simulink model "can2_comp_cmd_unpack"  (R2026b)
settings: Solver=VariableStepAuto
undefined symbols (not defined in the file or in its folder): P
libraries: simulink x1, svdutilitieslib x1
settings Model: Creator=aomar  LastModifiedBy=aomar

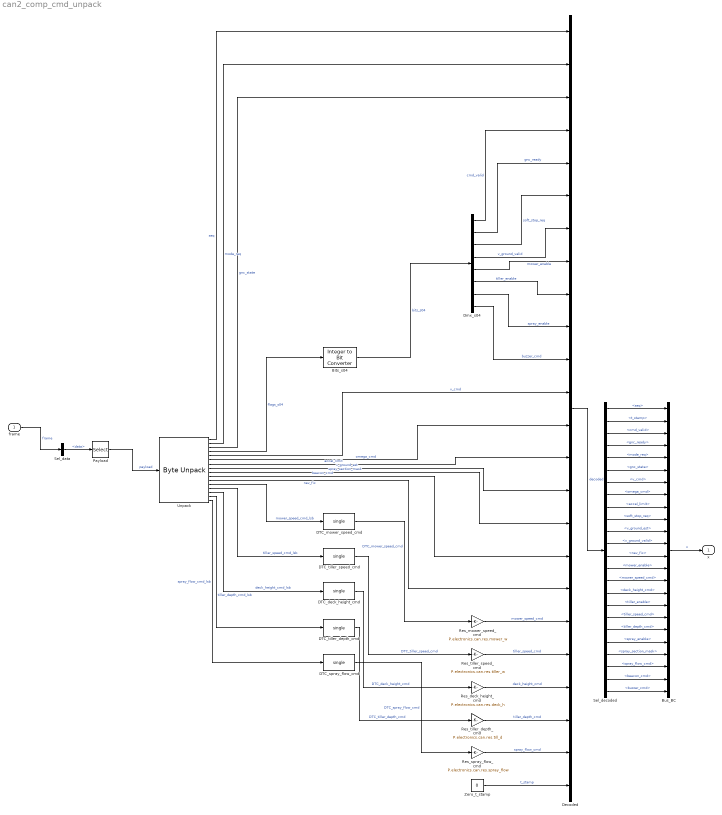
== system can2_comp_cmd_unpack ==
  frame : Inport  OutDataTypeStr=Bus: Bus_CanFrame64
  Bits_s04 : simulink/Logic and Bit Operations/Integer to Bit Converter  nbits=8  signedInputValues=Unsigned  bitOrder=LSB first  outDtype=boolean
      settings: LibrarySourceBlock=|
      | commutil2/Integer to Bit
      | Converter
  Bus_BC : BusCreator  Inputs=24  OutDataTypeStr=Bus: Bus_GncCmd  NonVirtualBus=on
      settings: InheritFromInputs=off
  DTC_deck_height_cmd : DataTypeConversion  OutDataTypeStr=single  SaturateOnIntegerOverflow=off  RndMeth=Floor
  DTC_mower_speed_cmd : DataTypeConversion  OutDataTypeStr=single  SaturateOnIntegerOverflow=off  RndMeth=Floor
  DTC_spray_flow_cmd : DataTypeConversion  OutDataTypeStr=single  SaturateOnIntegerOverflow=off  RndMeth=Floor
  DTC_tiller_depth_cmd : DataTypeConversion  OutDataTypeStr=single  SaturateOnIntegerOverflow=off  RndMeth=Floor
  DTC_tiller_speed_cmd : DataTypeConversion  OutDataTypeStr=single  SaturateOnIntegerOverflow=off  RndMeth=Floor
  Decoded : BusCreator  Inputs=24
  Dmx_s04 : Demux  Outputs=8
  Payload : Selector  InputPortWidth=64  IndexOptions=Index vector (dialog)  Indices=1:32  OutputSizes=1
  Res_deck_height_cmd : Gain  Gain=P.electronics.can.res.deck_h  OutDataTypeStr=single  ParamDataTypeStr=Inherit: Same as input
  Res_mower_speed_cmd : Gain  Gain=P.electronics.can.res.mower_w  OutDataTypeStr=single  ParamDataTypeStr=Inherit: Same as input
  Res_spray_flow_cmd : Gain  Gain=P.electronics.can.res.spray_flow  OutDataTypeStr=single  ParamDataTypeStr=Inherit: Same as input
  Res_tiller_depth_cmd : Gain  Gain=P.electronics.can.res.till_d  OutDataTypeStr=single  ParamDataTypeStr=Inherit: Same as input
  Res_tiller_speed_cmd : Gain  Gain=P.electronics.can.res.tiller_w  OutDataTypeStr=single  ParamDataTypeStr=Inherit: Same as input
  Sel_data : BusSelector  OutputSignals=data
  Sel_decoded : BusSelector  OutputSignals=seq,t_stamp,cmd_valid,gnc_ready,mode_req,gnc_state,v_cmd,omega_cmd,accel_limit,soft_stop_req,v_ground_est,v_ground_valid,nav_fix,mower_enable,mower_speed_cmd,deck_height_cmd,tiller_enable,tiller_speed_cmd,tiller_depth_cmd,spray_enable,spray_section_mask,spray_flow_cmd,beacon_cmd,buzzer_cmd
  Unpack : svdutilitieslib/Byte Unpack  dimensions={1,1,1,1,1,1,1,1,1,1,1,1,1,1,1,1}  datatypes={'uint8','uint8','uint8','uint8','single','single','single','single','uint16','uint8','uint8','uint16','uint16','uint8','uint8','uint16'}  byteAlign=1  blockPlatform=arduinoert
      settings: LibrarySourceBlock=mcblib/Signal Management/Byte Unpack
  Zero_t_stamp : Constant  Value=0  OutDataTypeStr=double  SampleTime=-1
  x : Outport  OutDataTypeStr=Bus: Bus_GncCmd
  wires:
  frame/1 -> Sel_data/1  "frame"
  Sel_data/1 -> Payload/1  "<data>"
  Payload/1 -> Unpack/1  "payload"
  Unpack/1 -> Decoded/1  "seq"
  Unpack/2 -> Decoded/2  "mode_req"
  Unpack/3 -> Decoded/3  "gnc_state"
  Unpack/4 -> Bits_s04/1  "flags_s04"
  Unpack/5 -> Decoded/12  "v_cmd"
  Unpack/6 -> Decoded/13  "omega_cmd"
  Unpack/7 -> Decoded/14  "accel_limit"
  Unpack/8 -> Decoded/15  "v_ground_est"
  Unpack/9 -> Decoded/16  "spray_section_mask"
  Unpack/10 -> Decoded/17  "beacon_cmd"
  Unpack/11 -> Decoded/18  "nav_fix"
  Unpack/12 -> DTC_mower_speed_cmd/1  "mower_speed_cmd_lsb"
  Unpack/13 -> DTC_tiller_speed_cmd/1  "tiller_speed_cmd_lsb"
  Unpack/14 -> DTC_deck_height_cmd/1  "deck_height_cmd_lsb"
  Unpack/15 -> DTC_tiller_depth_cmd/1  "tiller_depth_cmd_lsb"
  Unpack/16 -> DTC_spray_flow_cmd/1  "spray_flow_cmd_lsb"
  DTC_mower_speed_cmd/1 -> Res_mower_speed_cmd/1  "DTC_mower_speed_cmd"
  DTC_tiller_speed_cmd/1 -> Res_tiller_speed_cmd/1  "DTC_tiller_speed_cmd"
  DTC_deck_height_cmd/1 -> Res_deck_height_cmd/1  "DTC_deck_height_cmd"
  DTC_tiller_depth_cmd/1 -> Res_tiller_depth_cmd/1  "DTC_tiller_depth_cmd"
  DTC_spray_flow_cmd/1 -> Res_spray_flow_cmd/1  "DTC_spray_flow_cmd"
  Bits_s04/1 -> Dmx_s04/1  "bits_s04"
  Dmx_s04/1 -> Decoded/4  "cmd_valid"
  Dmx_s04/2 -> Decoded/5  "gnc_ready"
  Dmx_s04/3 -> Decoded/6  "soft_stop_req"
  Dmx_s04/4 -> Decoded/7  "v_ground_valid"
  Dmx_s04/5 -> Decoded/8  "mower_enable"
  Dmx_s04/6 -> Decoded/9  "tiller_enable"
  Dmx_s04/7 -> Decoded/10  "spray_enable"
  Dmx_s04/8 -> Decoded/11  "buzzer_cmd"
  Res_mower_speed_cmd/1 -> Decoded/19  "mower_speed_cmd"
  Res_tiller_speed_cmd/1 -> Decoded/20  "tiller_speed_cmd"
  Res_deck_height_cmd/1 -> Decoded/21  "deck_height_cmd"
  Res_tiller_depth_cmd/1 -> Decoded/22  "tiller_depth_cmd"
  Res_spray_flow_cmd/1 -> Decoded/23  "spray_flow_cmd"
  Zero_t_stamp/1 -> Decoded/24  "t_stamp"
  Decoded/1 -> Sel_decoded/1  "decoded"
  Sel_decoded/1 -> Bus_BC/1  "<seq>"
  Sel_decoded/2 -> Bus_BC/2  "<t_stamp>"
  Sel_decoded/3 -> Bus_BC/3  "<cmd_valid>"
  Sel_decoded/4 -> Bus_BC/4  "<gnc_ready>"
  Sel_decoded/5 -> Bus_BC/5  "<mode_req>"
  Sel_decoded/6 -> Bus_BC/6  "<gnc_state>"
  Sel_decoded/7 -> Bus_BC/7  "<v_cmd>"
  Sel_decoded/8 -> Bus_BC/8  "<omega_cmd>"
  Sel_decoded/9 -> Bus_BC/9  "<accel_limit>"
  Sel_decoded/10 -> Bus_BC/10  "<soft_stop_req>"
  Sel_decoded/11 -> Bus_BC/11  "<v_ground_est>"
  Sel_decoded/12 -> Bus_BC/12  "<v_ground_valid>"
  Sel_decoded/13 -> Bus_BC/13  "<nav_fix>"
  Sel_decoded/14 -> Bus_BC/14  "<mower_enable>"
  Sel_decoded/15 -> Bus_BC/15  "<mower_speed_cmd>"
  Sel_decoded/16 -> Bus_BC/16  "<deck_height_cmd>"
  Sel_decoded/17 -> Bus_BC/17  "<tiller_enable>"
  Sel_decoded/18 -> Bus_BC/18  "<tiller_speed_cmd>"
  Sel_decoded/19 -> Bus_BC/19  "<tiller_depth_cmd>"
  Sel_decoded/20 -> Bus_BC/20  "<spray_enable>"
  Sel_decoded/21 -> Bus_BC/21  "<spray_section_mask>"
  Sel_decoded/22 -> Bus_BC/22  "<spray_flow_cmd>"
  Sel_decoded/23 -> Bus_BC/23  "<beacon_cmd>"
  Sel_decoded/24 -> Bus_BC/24  "<buzzer_cmd>"
  Bus_BC/1 -> x/1  "x"
